simulink model "B2_manuel"  (R2022b)
settings: Solver=FixedStepDiscrete  StartTime=0.0  StopTime=45  FixedStep=Ts  RelTol=1e-3
values from neighbouring files (symbols this model uses):
  LUX_OFF = 2000    [build_B2_AutoHeadlamp.m]
  LUX_ON = 1000    [build_B2_AutoHeadlamp.m]
  T_OFF = 5    [build_B2_AutoHeadlamp.m]
  T_ON = 2    [build_B2_AutoHeadlamp.m]
  T_TUNNEL = 0.3    [build_B2_AutoHeadlamp.m]
  Ts = 0.01    [build_B2_AutoHeadlamp.m]    (also in build_B3_AHB.m)
settings Model: Creator=LENOVO  LastModifiedBy=LENOVO

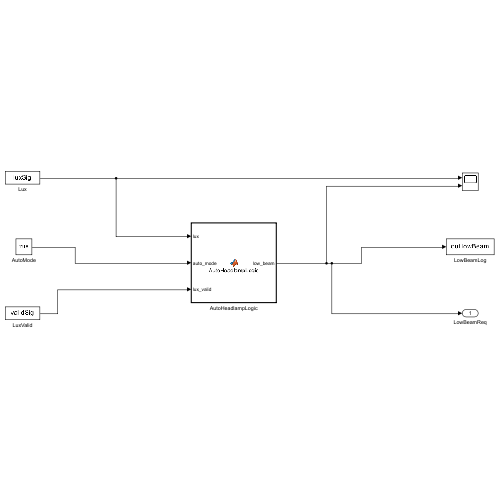
[thumbnail: Simulink's stored preview of the top-level diagram]
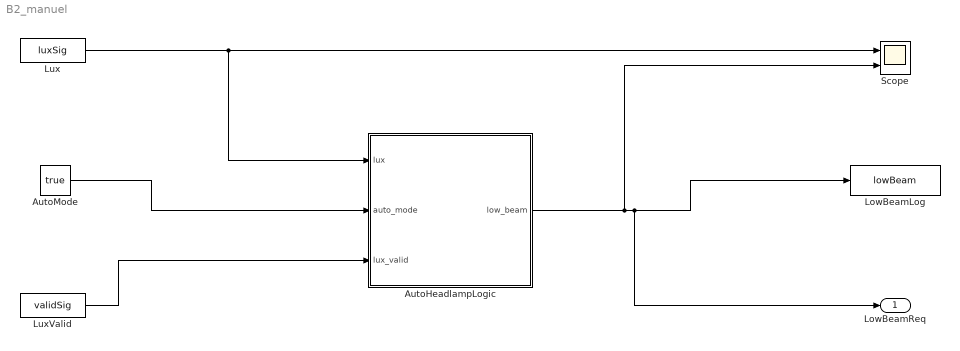
== system B2_manuel ==
  AutoHeadlampLogic : MATLAB Function  TreatAsAtomicUnit=on
  AutoMode : Constant  Value=true
  LowBeamLog : ToWorkspace  VariableName=lowBeam  SaveFormat=Timeseries  SampleTime=-1
  Lux : FromWorkspace  VariableName=luxSig  SampleTime=Ts  OutputAfterFinalValue=Holding final value
  LuxValid : FromWorkspace  VariableName=validSig  SampleTime=Ts  Interpolate=off  OutputAfterFinalValue=Holding final value
  Scope : Scope  NumInputPorts=2
  LowBeamReq : Outport
  wires:
  Lux/1 -> Scope/1, AutoHeadlampLogic/1(lux)
  AutoMode/1 -> AutoHeadlampLogic/2(auto_mode)
  LuxValid/1 -> AutoHeadlampLogic/3(lux_valid)
  AutoHeadlampLogic/1(low_beam) -> Scope/2, LowBeamReq/1, LowBeamLog/1

== matlab function B2_manuel/AutoHeadlampLogic ==
  data: lux input; low_beam output; auto_mode input; lux_valid input; LUX_ON parameter; LUX_OFF parameter; T_ON parameter; T_OFF parameter; T_TUNNEL parameter; Ts parameter
function low_beam = AutoHeadlampLogic(lux, auto_mode, lux_valid, LUX_ON, LUX_OFF, T_ON, T_OFF, T_TUNNEL, Ts)
%#codegen
% B2 - Auto Headlamp : allumage/extinction automatique avec hysteresis
persistent st cnt buf idx          % memoire conservee d'un pas a l'autre
N = 50;                            % 50 x 10 ms = 0,5 s d'historique
if isempty(st)                     % initialisation au 1er pas
    st = false; cnt = 0; buf = 10000*ones(1, N); idx = 1;
end
% --- Detection tunnel : chute > 80 % en 0,5 s
lux_past = buf(idx);
buf(idx) = lux;
idx = mod(idx, N) + 1;
tunnel = (lux < 0.2*lux_past) && (lux < LUX_ON);

% --- Logique principale
if ~auto_mode
    st = false; cnt = 0;           % pas en AUTO : B2 ne demande rien
elseif ~lux_valid
    st = true;  cnt = 0;           % capteur en defaut : etat sur
elseif ~st                         % feux eteints
    if lux < LUX_ON
        cnt = cnt + Ts;
        if (cnt > T_ON + Ts/2) || (tunnel && cnt > T_TUNNEL + Ts/2)
            st = true; cnt = 0;
        end
    else
        cnt = 0;                   % condition interrompue -> on recommence
    end
else                               % feux allumes
    if lux > LUX_OFF
        cnt = cnt + Ts;
        if cnt > T_OFF + Ts/2
            st = false; cnt = 0;
        end
    else
        cnt = 0;
    end
end
low_beam = st;
